simulink model "FullAssemblyMultibody"  (R2025b)
settings: Solver=ode23t  StartTime=0.0  StopTime=16  MaxStep=0.32  RelTol=0.01  AbsTol=1e-3
model workspace: external: MATLAB File E:\Apps\AutodeskInventor\University\MCT333_Design_of_Mechatronics_Systems_1\simscape_multibody_simulation\simulation\FullAssemblyMultibody_DataFile.m (data not in the file)
undefined symbols (not defined in the file or in its folder): smiData, X, Y, Z
libraries: sm_lib x160, Contact_Forces_Lib x46, nesl_utility x5, SignalEditorBlockLib x1
(part 2 of 5)

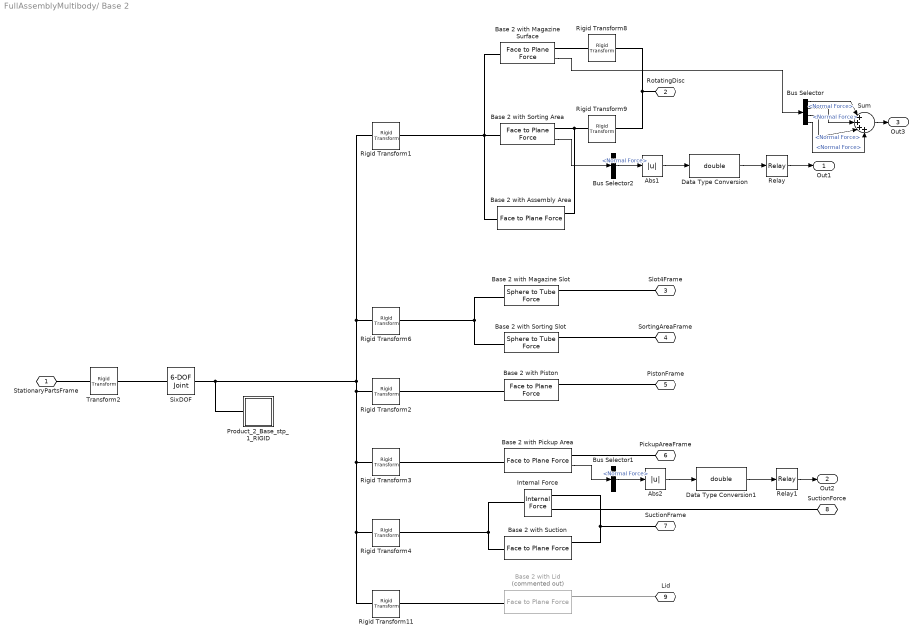
== system FullAssemblyMultibody/ Base 2 ==
  " Base 2 with Piston" : Contact_Forces_Lib/3D/Composite Forces/Face to Plane Force  PlaB_x=0.07  PlaB_y=0.07  PlaB_z=0  FacF_x=0.05  FacF_y=0.05  FacF_z=0.05  FacF_rSph=0.001  force_law_pla2pla=Linear  k_contact_pla2pla=1e4  b_contact_pla2pla=1e4  pen_full_damp_F_pla2pla=1e-4  pen_exponent_pla2pla=1  friction_law_pla2pla=Stick-Slip Continuous  mu_kinetic_pla2pla=0.1  mu_static_pla2pla=0.11  v_thr_pla2pla=0.01  vis_on_pla2pla=off  vis_opc_en_box2box=0  vis_len_plaLz=0.005  vis_clr=[0.9 0.2 0.2]  vis_opc=0.7
      settings: SourceProductName=Simscape Multibody Contact Forces Library
  Abs1 : Abs  SaturateOnIntegerOverflow=off
  Abs2 : Abs  SaturateOnIntegerOverflow=off
  Base 2 with Assembly Area : Contact_Forces_Lib/3D/Composite Forces/Face to Plane Force  PlaB_x=0.1  PlaB_y=0.1  PlaB_z=0  FacF_x=0.05  FacF_y=0.05  FacF_z=0.05  FacF_rSph=0.001  force_law_pla2pla=Linear  k_contact_pla2pla=1e4  b_contact_pla2pla=1e4  pen_full_damp_F_pla2pla=1e-4  pen_exponent_pla2pla=1  friction_law_pla2pla=Stick-Slip Continuous  mu_kinetic_pla2pla=0.1  mu_static_pla2pla=0.11  v_thr_pla2pla=0.01  vis_on_pla2pla=off  vis_opc_en_box2box=0  vis_len_plaLz=0.005  vis_clr=[0.9 0.2 0.2]  vis_opc=0.7
      settings: SourceProductName=Simscape Multibody Contact Forces Library
  Base 2 with Lid : Contact_Forces_Lib/3D/Composite Forces/Face to Plane Force  Commented=on  PlaB_x=0.1  PlaB_y=0.1  PlaB_z=0  FacF_x=0.05  FacF_y=0.05  FacF_z=0.05  FacF_rSph=0.001  force_law_pla2pla=Linear  k_contact_pla2pla=1e4  b_contact_pla2pla=1e4  pen_full_damp_F_pla2pla=1e-4  pen_exponent_pla2pla=1  friction_law_pla2pla=Stick-Slip Continuous  mu_kinetic_pla2pla=0.1  mu_static_pla2pla=0.11  v_thr_pla2pla=0.01  vis_on_pla2pla=off  vis_opc_en_box2box=0  vis_len_plaLz=0.005  vis_clr=[0.9 0.2 0.2]  vis_opc=0.7
      settings: SourceProductName=Simscape Multibody Contact Forces Library
  Base 2 with Magazine Slot : Contact_Forces_Lib/3D/Sphere to Tube Force  radius_sphere=0.05/2  radius_tube=0.070/2  d_tube=0.005  l_tube=.04  active_angle=[-180 180]  force_law=Linear  k_contact=100  b_contact=100  pen_full_damp_F=1e-4  pen_exponent=1  custom_param_1=1  custom_param_2=1  friction_law=Stick-Slip Continuous  mu_kinetic=0.1  mu_static=0.11  v_thr=0.001  vis_on=off  vis_opc_en=0  vis_len_tubBx=0.225*0.02  vis_clr=[0.9 0.2 0.2]  vis_opc=0.7
      settings: SourceProductName=Simscape Multibody Contact Forces Library
  Base 2 with Magazine Surface : Contact_Forces_Lib/3D/Composite Forces/Face to Plane Force  PlaB_x=0.4  PlaB_y=0.4  PlaB_z=0  FacF_x=0.04  FacF_y=0.04  FacF_z=0.05  FacF_rSph=0.001  force_law_pla2pla=Linear  k_contact_pla2pla=1e4  b_contact_pla2pla=1e4  pen_full_damp_F_pla2pla=1e-4  pen_exponent_pla2pla=1  friction_law_pla2pla=Stick-Slip Continuous  mu_kinetic_pla2pla=0.1  mu_static_pla2pla=0.11  v_thr_pla2pla=0.01  vis_on_pla2pla=on  vis_opc_en_box2box=0  vis_len_plaLz=0.005  vis_clr=[0.9 0.2 0.2]  vis_opc=0.7
      settings: SourceProductName=Simscape Multibody Contact Forces Library
  Base 2 with Pickup Area : Contact_Forces_Lib/3D/Composite Forces/Face to Plane Force  PlaB_x=0.1  PlaB_y=0.1  PlaB_z=0  FacF_x=0.05  FacF_y=0.05  FacF_z=0.05  FacF_rSph=0.001  force_law_pla2pla=Linear  k_contact_pla2pla=1e4  b_contact_pla2pla=1e4  pen_full_damp_F_pla2pla=1e-4  pen_exponent_pla2pla=1  friction_law_pla2pla=Stick-Slip Continuous  mu_kinetic_pla2pla=0.1  mu_static_pla2pla=0.11  v_thr_pla2pla=0.01  vis_on_pla2pla=off  vis_opc_en_box2box=0  vis_len_plaLz=0.005  vis_clr=[0.9 0.2 0.2]  vis_opc=0.7
      settings: SourceProductName=Simscape Multibody Contact Forces Library
  Base 2 with Sorting Area : Contact_Forces_Lib/3D/Composite Forces/Face to Plane Force  PlaB_x=1  PlaB_y=1  PlaB_z=0  FacF_x=0.04  FacF_y=0.04  FacF_z=0.05  FacF_rSph=0.001  force_law_pla2pla=Linear  k_contact_pla2pla=1e4  b_contact_pla2pla=1e4  pen_full_damp_F_pla2pla=1e-4  pen_exponent_pla2pla=1  friction_law_pla2pla=Stick-Slip Continuous  mu_kinetic_pla2pla=0.1  mu_static_pla2pla=0.11  v_thr_pla2pla=0.01  vis_on_pla2pla=off  vis_opc_en_box2box=0  vis_len_plaLz=0.005  vis_clr=[0.9 0.2 0.2]  vis_opc=0.7
      settings: SourceProductName=Simscape Multibody Contact Forces Library
  Base 2 with Sorting Slot : Contact_Forces_Lib/3D/Sphere to Tube Force  radius_sphere=0.05/2  radius_tube=0.070/2  d_tube=0.005  l_tube=.1  active_angle=[-180 180]  force_law=Linear  k_contact=100  b_contact=100  pen_full_damp_F=1e-4  pen_exponent=1  custom_param_1=1  custom_param_2=1  friction_law=Stick-Slip Continuous  mu_kinetic=0.1  mu_static=0.11  v_thr=0.001  vis_on=off  vis_opc_en=0  vis_len_tubBx=0.225*0.02  vis_clr=[0.9 0.2 0.2]  vis_opc=0.7
      settings: SourceProductName=Simscape Multibody Contact Forces Library
  Base 2 with Suction : Contact_Forces_Lib/3D/Composite Forces/Face to Plane Force  PlaB_x=0.05  PlaB_y=0.05  PlaB_z=0  FacF_x=0.04  FacF_y=0.04  FacF_z=0.05  FacF_rSph=0.001  force_law_pla2pla=Linear  k_contact_pla2pla=1e4  b_contact_pla2pla=1e4  pen_full_damp_F_pla2pla=1e-4  pen_exponent_pla2pla=1  friction_law_pla2pla=Stick-Slip Continuous  mu_kinetic_pla2pla=0.1  mu_static_pla2pla=0.11  v_thr_pla2pla=0.01  vis_on_pla2pla=off  vis_opc_en_box2box=0  vis_len_plaLz=0.005  vis_clr=[0.9 0.2 0.2]  vis_opc=0.7
      settings: SourceProductName=Simscape Multibody Contact Forces Library
  Bus Selector : BusSelector  OutputSignals=fz1.Normal Force,fz2.Normal Force,fz3.Normal Force,fz4.Normal Force
  Bus Selector1 : BusSelector  OutputSignals=fz1.Normal Force
  Bus Selector2 : BusSelector  OutputSignals=fz1.Normal Force
  Data Type Conversion : DataTypeConversion  OutDataTypeStr=double  SaturateOnIntegerOverflow=off  RndMeth=Floor
  Data Type Conversion1 : DataTypeConversion  OutDataTypeStr=double  SaturateOnIntegerOverflow=off  RndMeth=Floor
  Internal Force : sm_lib/Forces and Torques/Internal Force
  Product_2_Base_stp_1_RIGID : Subsystem
  Relay : Relay  OnSwitchValue=0.5  OffSwitchValue=0.005
  Relay1 : Relay  OnSwitchValue=0.5  OffSwitchValue=0.005
  Rigid Transform1 : sm_lib/Frames and Transforms/Rigid Transform  RotationMethod=StandardAxis  FollAlignAxisA=+X  BaseAlignAxisA=+Y  FollAlignAxisB=+Y  BaseAlignAxisB=+Z  RotationStandardAxis=+X  RotationAngle=90  RotationAngleUnits=deg  RotationArbitraryAxis=[0 0 1]  RotationSequenceAxes=FollowerAxes  RotationSequence=XYX  RotationSequenceAngles=[0 0 0]  RotationSequenceAnglesUnits=deg  RotationMatrix=[1 0 0;0 1 0;0 0 1]  Quaternion=[1 0 0 0]  TranslationMethod=StandardAxis  TranslationCartesianOffset=[0 0 0]  TranslationCartesianOffsetUnits=m  TranslationStandardAxis=-Y  TranslationStandardOffset=40  TranslationStandardOffsetUnits=mm  TranslationROffset=0  TranslationROffsetUnits=m  TranslationThetaOffset=0  TranslationThetaOffsetUnits=deg  TranslationZOffset=0  TranslationZOffsetUnits=m
  Rigid Transform11 : sm_lib/Frames and Transforms/Rigid Transform  RotationMethod=StandardAxis  FollAlignAxisA=+X  BaseAlignAxisA=+Y  FollAlignAxisB=+Y  BaseAlignAxisB=+Z  RotationStandardAxis=+X  RotationAngle=90  RotationAngleUnits=deg  RotationArbitraryAxis=[0 0 1]  RotationSequenceAxes=FollowerAxes  RotationSequence=XYX  RotationSequenceAngles=[0 0 0]  RotationSequenceAnglesUnits=deg  RotationMatrix=[1 0 0;0 1 0;0 0 1]  Quaternion=[1 0 0 0]  TranslationMethod=StandardAxis  TranslationCartesianOffset=[0 20 50]  TranslationCartesianOffsetUnits=mm  TranslationStandardAxis=-Y  TranslationStandardOffset=20  TranslationStandardOffsetUnits=mm  TranslationROffset=0  TranslationROffsetUnits=m  TranslationThetaOffset=0  TranslationThetaOffsetUnits=deg  TranslationZOffset=0  TranslationZOffsetUnits=m
  Rigid Transform2 : sm_lib/Frames and Transforms/Rigid Transform  RotationMethod=None  FollAlignAxisA=+X  BaseAlignAxisA=+Y  FollAlignAxisB=+Y  BaseAlignAxisB=+Z  RotationStandardAxis=+Z  RotationAngle=0  RotationAngleUnits=deg  RotationArbitraryAxis=[0 0 1]  RotationSequenceAxes=FollowerAxes  RotationSequence=XYX  RotationSequenceAngles=[0 0 0]  RotationSequenceAnglesUnits=deg  RotationMatrix=[1 0 0;0 1 0;0 0 1]  Quaternion=[1 0 0 0]  TranslationMethod=Cartesian  TranslationCartesianOffset=[0 20 50]  TranslationCartesianOffsetUnits=mm  TranslationStandardAxis=+Y  TranslationStandardOffset=50  TranslationStandardOffsetUnits=mm  TranslationROffset=0  TranslationROffsetUnits=m  TranslationThetaOffset=0  TranslationThetaOffsetUnits=deg  TranslationZOffset=0  TranslationZOffsetUnits=m
  Rigid Transform3 : sm_lib/Frames and Transforms/Rigid Transform  RotationMethod=None  FollAlignAxisA=+X  BaseAlignAxisA=+Y  FollAlignAxisB=+Y  BaseAlignAxisB=+Z  RotationStandardAxis=+X  RotationAngle=90  RotationAngleUnits=deg  RotationArbitraryAxis=[0 0 1]  RotationSequenceAxes=FollowerAxes  RotationSequence=XYX  RotationSequenceAngles=[0 0 0]  RotationSequenceAnglesUnits=deg  RotationMatrix=[1 0 0;0 1 0;0 0 1]  Quaternion=[1 0 0 0]  TranslationMethod=Cartesian  TranslationCartesianOffset=[0 20 50]  TranslationCartesianOffsetUnits=mm  TranslationStandardAxis=+Y  TranslationStandardOffset=50  TranslationStandardOffsetUnits=mm  TranslationROffset=0  TranslationROffsetUnits=m  TranslationThetaOffset=0  TranslationThetaOffsetUnits=deg  TranslationZOffset=0  TranslationZOffsetUnits=m
  Rigid Transform4 : sm_lib/Frames and Transforms/Rigid Transform  RotationMethod=StandardAxis  FollAlignAxisA=+X  BaseAlignAxisA=+Y  FollAlignAxisB=+Y  BaseAlignAxisB=+Z  RotationStandardAxis=+X  RotationAngle=90  RotationAngleUnits=deg  RotationArbitraryAxis=[0 0 1]  RotationSequenceAxes=FollowerAxes  RotationSequence=XYX  RotationSequenceAngles=[0 0 0]  RotationSequenceAnglesUnits=deg  RotationMatrix=[1 0 0;0 1 0;0 0 1]  Quaternion=[1 0 0 0]  TranslationMethod=StandardAxis  TranslationCartesianOffset=[0 20 50]  TranslationCartesianOffsetUnits=mm  TranslationStandardAxis=-Y  TranslationStandardOffset=10  TranslationStandardOffsetUnits=mm  TranslationROffset=0  TranslationROffsetUnits=m  TranslationThetaOffset=0  TranslationThetaOffsetUnits=deg  TranslationZOffset=0  TranslationZOffsetUnits=m
  Rigid Transform6 : sm_lib/Frames and Transforms/Rigid Transform  RotationMethod=None  FollAlignAxisA=+X  BaseAlignAxisA=+Y  FollAlignAxisB=+Y  BaseAlignAxisB=+Z  RotationStandardAxis=+Z  RotationAngle=0  RotationAngleUnits=deg  RotationArbitraryAxis=[0 0 1]  RotationSequenceAxes=FollowerAxes  RotationSequence=XYX  RotationSequenceAngles=[0 0 0]  RotationSequenceAnglesUnits=deg  RotationMatrix=[1 0 0;0 1 0;0 0 1]  Quaternion=[1 0 0 0]  TranslationMethod=StandardAxis  TranslationCartesianOffset=[0 0 0]  TranslationCartesianOffsetUnits=m  TranslationStandardAxis=+Y  TranslationStandardOffset=15  TranslationStandardOffsetUnits=mm  TranslationROffset=0  TranslationROffsetUnits=m  TranslationThetaOffset=0  TranslationThetaOffsetUnits=deg  TranslationZOffset=0  TranslationZOffsetUnits=m
  Rigid Transform8 : sm_lib/Frames and Transforms/Rigid Transform  RotationMethod=None  FollAlignAxisA=+X  BaseAlignAxisA=+Y  FollAlignAxisB=+Y  BaseAlignAxisB=+Z  RotationStandardAxis=+Z  RotationAngle=0  RotationAngleUnits=deg  RotationArbitraryAxis=[0 0 1]  RotationSequenceAxes=FollowerAxes  RotationSequence=XYX  RotationSequenceAngles=[0 0 0]  RotationSequenceAnglesUnits=deg  RotationMatrix=[1 0 0;0 1 0;0 0 1]  Quaternion=[1 0 0 0]  TranslationMethod=StandardAxis  TranslationCartesianOffset=[0 0 0]  TranslationCartesianOffsetUnits=m  TranslationStandardAxis=-X  TranslationStandardOffset=225  TranslationStandardOffsetUnits=mm  TranslationROffset=0  TranslationROffsetUnits=m  TranslationThetaOffset=0  TranslationThetaOffsetUnits=deg  TranslationZOffset=0  TranslationZOffsetUnits=m
  Rigid Transform9 : sm_lib/Frames and Transforms/Rigid Transform  RotationMethod=None  FollAlignAxisA=+X  BaseAlignAxisA=+Y  FollAlignAxisB=+Y  BaseAlignAxisB=+Z  RotationStandardAxis=+Z  RotationAngle=0  RotationAngleUnits=deg  RotationArbitraryAxis=[0 0 1]  RotationSequenceAxes=FollowerAxes  RotationSequence=XYX  RotationSequenceAngles=[0 0 0]  RotationSequenceAnglesUnits=deg  RotationMatrix=[1 0 0;0 1 0;0 0 1]  Quaternion=[1 0 0 0]  TranslationMethod=StandardAxis  TranslationCartesianOffset=[0 0 0]  TranslationCartesianOffsetUnits=m  TranslationStandardAxis=+Z  TranslationStandardOffset=120  TranslationStandardOffsetUnits=mm  TranslationROffset=0  TranslationROffsetUnits=m  TranslationThetaOffset=0  TranslationThetaOffsetUnits=deg  TranslationZOffset=0  TranslationZOffsetUnits=m
  SixDOF : sm_lib/Joints/6-DOF Joint  JointMode=Normal  CompositeWrenchDir=FollowerOnBase  CompositeWrenchFrame=BaseFrame  SenseConstraintForce=off  SenseConstraintTorque=off  SenseTotalForce=off  SenseTotalTorque=off  PxPositionTargetSpecify=off  PxPositionTargetPriority=High  PxPositionTargetValue=0  PxPositionTargetValueUnits=m  PxVelocityTargetSpecify=off  PxVelocityTargetPriority=High  PxVelocityTargetValue=0  PxVelocityTargetValueUnits=m/s  PxEquilibriumPosition=0  PxEquilibriumPositionUnits=m  PxSpringStiffness=0  PxSpringStiffnessUnits=N/m  PxDampingCoefficient=0  PxDampingCoefficientUnits=N/(m/s)  PxLowerLimitSpecify=off  PxLowerLimitBound=-1  PxLowerLimitBoundUnits=m  PxLowerLimitStiffness=1e6  PxLowerLimitStiffnessUnits=N/m  PxLowerLimitDamping=1e3  PxLowerLimitDampingUnits=N/(m/s)  PxLowerLimitTransitionRegionWidth=1e-4  PxLowerLimitTransitionRegionWidthUnits=m  PxUpperLimitSpecify=off  PxUpperLimitBound=1  PxUpperLimitBoundUnits=m  PxUpperLimitStiffness=1e6  PxUpperLimitStiffnessUnits=N/m  PxUpperLimitDamping=1e3  PxUpperLimitDampingUnits=N/(m/s)  PxUpperLimitTransitionRegionWidth=1e-4  PxUpperLimitTransitionRegionWidthUnits=m  PxTorqueActuationMode=NoTorque  PxMotionActuationMode=ComputedMotion  PxSensePosition=off  PxSenseVelocity=off  PxSenseAcceleration=off  PxSenseTorqueForce=off  PxSenseLowerLimitTorqueForce=off  PxSenseUpperLimitTorqueForce=off  PyPositionTargetSpecify=on  PyPositionTargetPriority=High  PyPositionTargetValue=30  PyPositionTargetValueUnits=mm  PyVelocityTargetSpecify=off  PyVelocityTargetPriority=High  PyVelocityTargetValue=0  PyVelocityTargetValueUnits=m/s  PyEquilibriumPosition=0  PyEquilibriumPositionUnits=m  PySpringStiffness=0  PySpringStiffnessUnits=N/m  PyDampingCoefficient=0  PyDampingCoefficientUnits=N/(m/s)  PyLowerLimitSpecify=off  PyLowerLimitBound=-1  PyLowerLimitBoundUnits=m  PyLowerLimitStiffness=1e6  PyLowerLimitStiffnessUnits=N/m  PyLowerLimitDamping=1e3  PyLowerLimitDampingUnits=N/(m/s)  PyLowerLimitTransitionRegionWidth=1e-4  PyLowerLimitTransitionRegionWidthUnits=m  PyUpperLimitSpecify=off  PyUpperLimitBound=1  PyUpperLimitBoundUnits=m  PyUpperLimitStiffness=1e6  PyUpperLimitStiffnessUnits=N/m  PyUpperLimitDamping=1e3  PyUpperLimitDampingUnits=N/(m/s)  PyUpperLimitTransitionRegionWidth=1e-4  PyUpperLimitTransitionRegionWidthUnits=m  PyTorqueActuationMode=NoTorque  PyMotionActuationMode=ComputedMotion  PySensePosition=off  PySenseVelocity=off  PySenseAcceleration=off  PySenseTorqueForce=off  PySenseLowerLimitTorqueForce=off  PySenseUpperLimitTorqueForce=off  PzPositionTargetSpecify=off  PzPositionTargetPriority=High  PzPositionTargetValue=0  PzPositionTargetValueUnits=m  PzVelocityTargetSpecify=off  PzVelocityTargetPriority=High  PzVelocityTargetValue=0  PzVelocityTargetValueUnits=m/s  PzEquilibriumPosition=0  PzEquilibriumPositionUnits=m  PzSpringStiffness=0  PzSpringStiffnessUnits=N/m  PzDampingCoefficient=0  PzDampingCoefficientUnits=N/(m/s)  PzLowerLimitSpecify=off  PzLowerLimitBound=-1  PzLowerLimitBoundUnits=m  PzLowerLimitStiffness=1e6  PzLowerLimitStiffnessUnits=N/m  PzLowerLimitDamping=1e3  PzLowerLimitDampingUnits=N/(m/s)  PzLowerLimitTransitionRegionWidth=1e-4  PzLowerLimitTransitionRegionWidthUnits=m  PzUpperLimitSpecify=off  PzUpperLimitBound=1  PzUpperLimitBoundUnits=m  PzUpperLimitStiffness=1e6  PzUpperLimitStiffnessUnits=N/m  PzUpperLimitDamping=1e3  PzUpperLimitDampingUnits=N/(m/s)  PzUpperLimitTransitionRegionWidth=1e-4  PzUpperLimitTransitionRegionWidthUnits=m  PzTorqueActuationMode=NoTorque  PzMotionActuationMode=ComputedMotion  PzSensePosition=off  PzSenseVelocity=off  PzSenseAcceleration=off  PzSenseTorqueForce=off  PzSenseLowerLimitTorqueForce=off  PzSenseUpperLimitTorqueForce=off  SphPositionTargetSpecify=off  SphPositionTargetPriority=High  SphPositionTargetRotationMethod=None  SphPositionTargetFollAlignAxisA=+X  SphPositionTargetBaseAlignAxisA=+Y  SphPositionTargetFollAlignAxisB=+Y  SphPositionTargetBaseAlignAxisB=+Z  SphPositionTargetRotationStandardAxis=+Z  SphPositionTargetRotationAngle=0  SphPositionTargetRotationAngleUnits=deg  SphPositionTargetRotationArbitraryAxis=[0 0 1]  SphPositionTargetRotationSequenceAxes=FollowerAxes  SphPositionTargetRotationSequence=XYX  SphPositionTargetRotationSequenceAngles=[0 0 0]  SphPositionTargetRotationSequenceAnglesUnits=deg  SphPositionTargetRotationMatrix=[1 0 0;0 1 0;0 0 1]  SphPositionTargetQuaternion=[1 0 0 0]  SphVelocityTargetSpecify=off  SphVelocityTargetPriority=High  SphVelocityTargetValue=[0 0 0]  SphVelocityTargetValueUnits=deg/s  SphVelocityTargetInFollowerFrame=on  SphEqPosRotationMethod=None  SphEqPosFollAlignAxisA=+X  SphEqPosBaseAlignAxisA=+Y  SphEqPosFollAlignAxisB=+Y  SphEqPosBaseAlignAxisB=+Z  SphEqPosRotationStandardAxis=+Z  SphEqPosRotationAngle=0  SphEqPosRotationAngleUnits=deg  SphEqPosRotationArbitraryAxis=[0 0 1]  SphEqPosRotationSequenceAxes=FollowerAxes  SphEqPosRotationSequence=XYX  SphEqPosRotationSequenceAngles=[0 0 0]  SphEqPosRotationSequenceAnglesUnits=deg  SphEqPosRotationMatrix=[1 0 0;0 1 0;0 0 1]  SphEqPosQuaternion=[1 0 0 0]  SphSpringStiffness=0  SphSpringStiffnessUnits=N*m/deg  SphDampingCoefficient=0  SphDampingCoefficientUnits=N*m/(deg/s)  SphLowerLimitSpecify=off  SphLowerLimitBound=15  SphLowerLimitBoundUnits=deg  SphLowerLimitStiffness=1e4  SphLowerLimitStiffnessUnits=N*m/deg  SphLowerLimitDamping=10  SphLowerLimitDampingUnits=N*m/(deg/s)  SphLowerLimitTransitionRegionWidth=0.1  SphLowerLimitTransitionRegionWidthUnits=deg  SphUpperLimitSpecify=off  SphUpperLimitBound=45  SphUpperLimitBoundUnits=deg  SphUpperLimitStiffness=1e4  SphUpperLimitStiffnessUnits=N*m/deg  SphUpperLimitDamping=10  SphUpperLimitDampingUnits=N*m/(deg/s)  SphUpperLimitTransitionRegionWidth=0.1  SphUpperLimitTransitionRegionWidthUnits=deg  SphTorqueActuationMode=NoTorque  SphActuateTorqueX=off  SphActuateTorqueY=off  SphActuateTorqueZ=off  SphActuateTorque=off  SphActuationFrame=BaseFrame  SphSensePosition=off  SphSenseVelocityX=off  SphSenseVelocityY=off  SphSenseVelocityZ=off  SphSenseVelocity=off  SphSenseAccelerationX=off  SphSenseAccelerationY=off  SphSenseAccelerationZ=off  SphSenseAcceleration=off  SphSenseLowerLimitTorqueMag=off  SphSenseUpperLimitTorqueMag=off  SphSensingFrame=FollowerFrame
  Sum : Sum  Inputs=|++++
  Transform2 : sm_lib/Frames and Transforms/Rigid Transform  RotationMethod=ArbitraryAxis  FollAlignAxisA=+X  BaseAlignAxisA=+Y  FollAlignAxisB=+Y  BaseAlignAxisB=+Z  RotationStandardAxis=+Z  RotationAngle=smiData.RigidTransform(31).angle  RotationAngleUnits=rad  RotationArbitraryAxis=smiData.RigidTransform(31).axis  RotationSequenceAxes=FollowerAxes  RotationSequence=XYX  RotationSequenceAngles=[0 0 0]  RotationSequenceAnglesUnits=deg  RotationMatrix=[1 0 0;0 1 0;0 0 1]  Quaternion=[1 0 0 0]  TranslationMethod=Cartesian  TranslationCartesianOffset=smiData.RigidTransform(31).translation  TranslationCartesianOffsetUnits=mm  TranslationStandardAxis=+Z  TranslationStandardOffset=0  TranslationStandardOffsetUnits=m  TranslationROffset=0  TranslationROffsetUnits=m  TranslationThetaOffset=0  TranslationThetaOffsetUnits=deg  TranslationZOffset=0  TranslationZOffsetUnits=m
  StationaryPartsFrame : PMIOPort  Side=Left
  RotatingDisc : PMIOPort  Port=2  Side=Left
  Slot4Frame : PMIOPort  Port=3  Side=Left
  SortingAreaFrame : PMIOPort  Port=4  Side=Left
  PistonFrame : PMIOPort  Port=5  Side=Left
  PickupAreaFrame : PMIOPort  Port=6  Side=Left
  SuctionFrame : PMIOPort  Port=7  Side=Left
  " SuctionForce" : PMIOPort  Port=8  Side=Left
  Lid : PMIOPort  Port=9  Side=Left
  Out1 : Outport
  Out2 : Outport  Port=2
  Out3 : Outport  Port=3
  wires:
  Base 2 with Pickup Area/1 -> Bus Selector1/1
  Base 2 with Sorting Area/1 -> Bus Selector2/1
  Bus Selector2/1 -> Abs1/1  "<Normal Force>"
  Abs1/1 -> Data Type Conversion/1
  Relay/1 -> Out1/1
  Data Type Conversion/1 -> Relay/1
  Bus Selector1/1 -> Abs2/1  "<Normal Force>"
  Abs2/1 -> Data Type Conversion1/1
  Data Type Conversion1/1 -> Relay1/1
  Relay1/1 -> Out2/1
  Base 2 with Magazine Surface/1 -> Bus Selector/1
  Sum/1 -> Out3/1
  Bus Selector/2 -> Sum/2  "<Normal Force>"
  Bus Selector/4 -> Sum/4  "<Normal Force>"
  Bus Selector/1 -> Sum/1  "<Normal Force>"
  Bus Selector/3 -> Sum/3  "<Normal Force>"
  connections:
  Base 2 with Sorting Slot/RConn1 -- SortingAreaFrame/RConn1
  Transform2/LConn1 -- StationaryPartsFrame/RConn1
  Slot4Frame/RConn1 -- Base 2 with Magazine Slot/RConn1
  Rigid Transform8/LConn1 -- RotatingDisc/RConn1 -- Rigid Transform9/LConn1
  Base 2 with Sorting Area/RConn1 -- Rigid Transform9/RConn1 -- Base 2 with Assembly Area/RConn1
  Base 2 with Magazine Slot/LConn1 -- Rigid Transform6/RConn1 -- Base 2 with Sorting Slot/LConn1
  Base 2 with Magazine Surface/RConn1 -- Rigid Transform8/RConn1
  Rigid Transform11/LConn1 -- Rigid Transform4/LConn1 -- Rigid Transform3/LConn1 -- Rigid Transform2/LConn1 -- Rigid Transform6/LConn1 -- Rigid Transform1/LConn1 -- Product_2_Base_stp_1_RIGID/LConn1 -- SixDOF/RConn1
  Transform2/RConn1 -- SixDOF/LConn1
  " Base 2 with Piston"/RConn1 -- PistonFrame/RConn1
  Rigid Transform3/RConn1 -- Base 2 with Pickup Area/LConn1
  PickupAreaFrame/RConn1 -- Base 2 with Pickup Area/RConn1
  Rigid Transform2/RConn1 -- " Base 2 with Piston"/LConn1
  Rigid Transform4/RConn1 -- Base 2 with Suction/LConn1 -- Internal Force/RConn1
  Base 2 with Suction/RConn1 -- SuctionFrame/RConn1 -- Internal Force/LConn1
  Rigid Transform11/RConn1 -- Base 2 with Lid/LConn1
  Base 2 with Lid/RConn1 -- Lid/RConn1
  " SuctionForce"/RConn1 -- Internal Force/LConn2
  Base 2 with Magazine Surface/LConn1 -- Rigid Transform1/RConn1 -- Base 2 with Sorting Area/LConn1 -- Base 2 with Assembly Area/LConn1

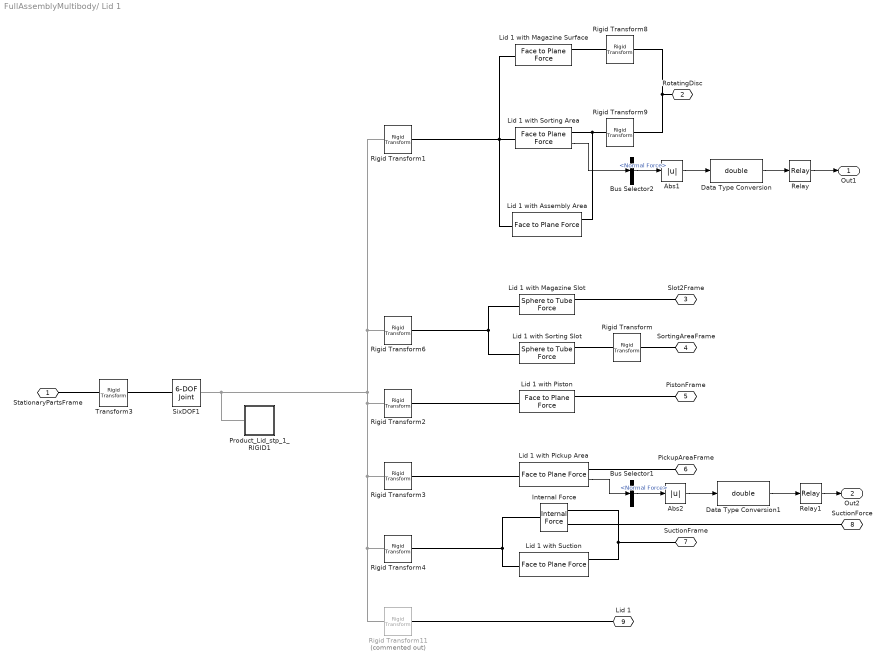
== system FullAssemblyMultibody/ Lid 1 ==
  " Lid 1 with Piston" : Contact_Forces_Lib/3D/Composite Forces/Face to Plane Force  PlaB_x=0.07  PlaB_y=0.07  PlaB_z=0  FacF_x=0.05  FacF_y=0.05  FacF_z=0.05  FacF_rSph=0.001  force_law_pla2pla=Linear  k_contact_pla2pla=1e4  b_contact_pla2pla=1e4  pen_full_damp_F_pla2pla=1e-4  pen_exponent_pla2pla=1  friction_law_pla2pla=Stick-Slip Continuous  mu_kinetic_pla2pla=0.1  mu_static_pla2pla=0.11  v_thr_pla2pla=0.01  vis_on_pla2pla=off  vis_opc_en_box2box=0  vis_len_plaLz=0.005  vis_clr=[0.9 0.2 0.2]  vis_opc=0.7
      settings: SourceProductName=Simscape Multibody Contact Forces Library
  Abs1 : Abs  SaturateOnIntegerOverflow=off
  Abs2 : Abs  SaturateOnIntegerOverflow=off
  Bus Selector1 : BusSelector  OutputSignals=fz1.Normal Force
  Bus Selector2 : BusSelector  OutputSignals=fz1.Normal Force
  Data Type Conversion : DataTypeConversion  OutDataTypeStr=double  SaturateOnIntegerOverflow=off  RndMeth=Floor
  Data Type Conversion1 : DataTypeConversion  OutDataTypeStr=double  SaturateOnIntegerOverflow=off  RndMeth=Floor
  Internal Force : sm_lib/Forces and Torques/Internal Force
  Lid 1 with Assembly Area : Contact_Forces_Lib/3D/Composite Forces/Face to Plane Force  PlaB_x=0.1  PlaB_y=0.1  PlaB_z=0  FacF_x=0.05  FacF_y=0.05  FacF_z=0.05  FacF_rSph=0.001  force_law_pla2pla=Linear  k_contact_pla2pla=1e4  b_contact_pla2pla=1e4  pen_full_damp_F_pla2pla=1e-4  pen_exponent_pla2pla=1  friction_law_pla2pla=Stick-Slip Continuous  mu_kinetic_pla2pla=0.1  mu_static_pla2pla=0.11  v_thr_pla2pla=0.01  vis_on_pla2pla=off  vis_opc_en_box2box=0  vis_len_plaLz=0.005  vis_clr=[0.9 0.2 0.2]  vis_opc=0.7
      settings: SourceProductName=Simscape Multibody Contact Forces Library
  Lid 1 with Magazine Slot : Contact_Forces_Lib/3D/Sphere to Tube Force  radius_sphere=0.05/2  radius_tube=0.070/2  d_tube=0.005  l_tube=.04  active_angle=[-180 180]  force_law=Linear  k_contact=100  b_contact=100  pen_full_damp_F=1e-4  pen_exponent=1  custom_param_1=1  custom_param_2=1  friction_law=Stick-Slip Continuous  mu_kinetic=0.1  mu_static=0.11  v_thr=0.001  vis_on=off  vis_opc_en=0  vis_len_tubBx=0.225*0.02  vis_clr=[0.9 0.2 0.2]  vis_opc=0.7
      settings: SourceProductName=Simscape Multibody Contact Forces Library
  Lid 1 with Magazine Surface : Contact_Forces_Lib/3D/Composite Forces/Face to Plane Force  PlaB_x=0.4  PlaB_y=0.4  PlaB_z=0  FacF_x=0.04  FacF_y=0.04  FacF_z=0.05  FacF_rSph=0.001  force_law_pla2pla=Linear  k_contact_pla2pla=1e4  b_contact_pla2pla=1e4  pen_full_damp_F_pla2pla=1e-4  pen_exponent_pla2pla=1  friction_law_pla2pla=Stick-Slip Continuous  mu_kinetic_pla2pla=0.1  mu_static_pla2pla=0.11  v_thr_pla2pla=0.01  vis_on_pla2pla=off  vis_opc_en_box2box=0  vis_len_plaLz=0.005  vis_clr=[0.9 0.2 0.2]  vis_opc=0.7
      settings: SourceProductName=Simscape Multibody Contact Forces Library
  Lid 1 with Pickup Area : Contact_Forces_Lib/3D/Composite Forces/Face to Plane Force  PlaB_x=0.1  PlaB_y=0.1  PlaB_z=0  FacF_x=0.05  FacF_y=0.05  FacF_z=0.05  FacF_rSph=0.001  force_law_pla2pla=Linear  k_contact_pla2pla=1e4  b_contact_pla2pla=1e4  pen_full_damp_F_pla2pla=1e-4  pen_exponent_pla2pla=1  friction_law_pla2pla=Stick-Slip Continuous  mu_kinetic_pla2pla=0.1  mu_static_pla2pla=0.11  v_thr_pla2pla=0.01  vis_on_pla2pla=off  vis_opc_en_box2box=0  vis_len_plaLz=0.005  vis_clr=[0.9 0.2 0.2]  vis_opc=0.7
      settings: SourceProductName=Simscape Multibody Contact Forces Library
  Lid 1 with Sorting Area : Contact_Forces_Lib/3D/Composite Forces/Face to Plane Force  PlaB_x=1  PlaB_y=1  PlaB_z=0  FacF_x=0.04  FacF_y=0.04  FacF_z=0.05  FacF_rSph=0.001  force_law_pla2pla=Linear  k_contact_pla2pla=1e4  b_contact_pla2pla=1e4  pen_full_damp_F_pla2pla=1e-4  pen_exponent_pla2pla=1  friction_law_pla2pla=Stick-Slip Continuous  mu_kinetic_pla2pla=0.1  mu_static_pla2pla=0.11  v_thr_pla2pla=0.01  vis_on_pla2pla=off  vis_opc_en_box2box=0  vis_len_plaLz=0.005  vis_clr=[0.9 0.2 0.2]  vis_opc=0.7
      settings: SourceProductName=Simscape Multibody Contact Forces Library
  Lid 1 with Sorting Slot : Contact_Forces_Lib/3D/Sphere to Tube Force  radius_sphere=0.05/2  radius_tube=0.055/2  d_tube=0.005  l_tube=.11  active_angle=[-180 180]  force_law=Linear  k_contact=100  b_contact=100  pen_full_damp_F=1e-4  pen_exponent=1  custom_param_1=1  custom_param_2=1  friction_law=Stick-Slip Continuous  mu_kinetic=0.1  mu_static=0.11  v_thr=0.001  vis_on=off  vis_opc_en=0  vis_len_tubBx=0.225*0.02  vis_clr=[0.9 0.2 0.2]  vis_opc=0.7
      settings: SourceProductName=Simscape Multibody Contact Forces Library
  Lid 1 with Suction : Contact_Forces_Lib/3D/Composite Forces/Face to Plane Force  PlaB_x=0.05  PlaB_y=0.05  PlaB_z=0  FacF_x=0.04  FacF_y=0.04  FacF_z=0.05  FacF_rSph=0.001  force_law_pla2pla=Linear  k_contact_pla2pla=1e4  b_contact_pla2pla=1e4  pen_full_damp_F_pla2pla=1e-4  pen_exponent_pla2pla=1  friction_law_pla2pla=Stick-Slip Continuous  mu_kinetic_pla2pla=0.1  mu_static_pla2pla=0.11  v_thr_pla2pla=0.01  vis_on_pla2pla=off  vis_opc_en_box2box=0  vis_len_plaLz=0.005  vis_clr=[0.9 0.2 0.2]  vis_opc=0.7
      settings: SourceProductName=Simscape Multibody Contact Forces Library
  Product_Lid_stp_1_RIGID1 : Subsystem
  Relay : Relay  OnSwitchValue=0.5  OffSwitchValue=0.005
  Relay1 : Relay  OnSwitchValue=0.5  OffSwitchValue=0.005
  Rigid Transform : sm_lib/Frames and Transforms/Rigid Transform  RotationMethod=None  FollAlignAxisA=+X  BaseAlignAxisA=+Y  FollAlignAxisB=+Y  BaseAlignAxisB=+Z  RotationStandardAxis=+Z  RotationAngle=0  RotationAngleUnits=deg  RotationArbitraryAxis=[0 0 1]  RotationSequenceAxes=FollowerAxes  RotationSequence=XYX  RotationSequenceAngles=[0 0 0]  RotationSequenceAnglesUnits=deg  RotationMatrix=[1 0 0;0 1 0;0 0 1]  Quaternion=[1 0 0 0]  TranslationMethod=StandardAxis  TranslationCartesianOffset=[0 0 0]  TranslationCartesianOffsetUnits=m  TranslationStandardAxis=+Z  TranslationStandardOffset=20  TranslationStandardOffsetUnits=mm  TranslationROffset=0  TranslationROffsetUnits=m  TranslationThetaOffset=0  TranslationThetaOffsetUnits=deg  TranslationZOffset=0  TranslationZOffsetUnits=m
  Rigid Transform1 : sm_lib/Frames and Transforms/Rigid Transform  RotationMethod=StandardAxis  FollAlignAxisA=+X  BaseAlignAxisA=+Y  FollAlignAxisB=+Y  BaseAlignAxisB=+Z  RotationStandardAxis=+X  RotationAngle=90  RotationAngleUnits=deg  RotationArbitraryAxis=[0 0 1]  RotationSequenceAxes=FollowerAxes  RotationSequence=XYX  RotationSequenceAngles=[0 0 0]  RotationSequenceAnglesUnits=deg  RotationMatrix=[1 0 0;0 1 0;0 0 1]  Quaternion=[1 0 0 0]  TranslationMethod=StandardAxis  TranslationCartesianOffset=[0 0 0]  TranslationCartesianOffsetUnits=m  TranslationStandardAxis=-Y  TranslationStandardOffset=40  TranslationStandardOffsetUnits=mm  TranslationROffset=0  TranslationROffsetUnits=m  TranslationThetaOffset=0  TranslationThetaOffsetUnits=deg  TranslationZOffset=0  TranslationZOffsetUnits=m
  Rigid Transform11 : sm_lib/Frames and Transforms/Rigid Transform  Commented=on  RotationMethod=StandardAxis  FollAlignAxisA=+X  BaseAlignAxisA=+Y  FollAlignAxisB=+Y  BaseAlignAxisB=+Z  RotationStandardAxis=+X  RotationAngle=90  RotationAngleUnits=deg  RotationArbitraryAxis=[0 0 1]  RotationSequenceAxes=FollowerAxes  RotationSequence=XYX  RotationSequenceAngles=[0 0 0]  RotationSequenceAnglesUnits=deg  RotationMatrix=[1 0 0;0 1 0;0 0 1]  Quaternion=[1 0 0 0]  TranslationMethod=StandardAxis  TranslationCartesianOffset=[0 20 50]  TranslationCartesianOffsetUnits=mm  TranslationStandardAxis=-Y  TranslationStandardOffset=20  TranslationStandardOffsetUnits=mm  TranslationROffset=0  TranslationROffsetUnits=m  TranslationThetaOffset=0  TranslationThetaOffsetUnits=deg  TranslationZOffset=0  TranslationZOffsetUnits=m
  Rigid Transform2 : sm_lib/Frames and Transforms/Rigid Transform  RotationMethod=StandardAxis  FollAlignAxisA=+X  BaseAlignAxisA=+Y  FollAlignAxisB=+Y  BaseAlignAxisB=+Z  RotationStandardAxis=+Z  RotationAngle=90  RotationAngleUnits=deg  RotationArbitraryAxis=[0 0 1]  RotationSequenceAxes=FollowerAxes  RotationSequence=XYX  RotationSequenceAngles=[0 0 0]  RotationSequenceAnglesUnits=deg  RotationMatrix=[1 0 0;0 1 0;0 0 1]  Quaternion=[1 0 0 0]  TranslationMethod=Cartesian  TranslationCartesianOffset=[0 20 70]  TranslationCartesianOffsetUnits=mm  TranslationStandardAxis=+Y  TranslationStandardOffset=50  TranslationStandardOffsetUnits=mm  TranslationROffset=0  TranslationROffsetUnits=m  TranslationThetaOffset=0  TranslationThetaOffsetUnits=deg  TranslationZOffset=0  TranslationZOffsetUnits=m
  Rigid Transform3 : sm_lib/Frames and Transforms/Rigid Transform  RotationMethod=None  FollAlignAxisA=+X  BaseAlignAxisA=+Y  FollAlignAxisB=+Y  BaseAlignAxisB=+Z  RotationStandardAxis=+X  RotationAngle=90  RotationAngleUnits=deg  RotationArbitraryAxis=[0 0 1]  RotationSequenceAxes=FollowerAxes  RotationSequence=XYX  RotationSequenceAngles=[0 0 0]  RotationSequenceAnglesUnits=deg  RotationMatrix=[1 0 0;0 1 0;0 0 1]  Quaternion=[1 0 0 0]  TranslationMethod=Cartesian  TranslationCartesianOffset=[0 20 50]  TranslationCartesianOffsetUnits=mm  TranslationStandardAxis=+Y  TranslationStandardOffset=50  TranslationStandardOffsetUnits=mm  TranslationROffset=0  TranslationROffsetUnits=m  TranslationThetaOffset=0  TranslationThetaOffsetUnits=deg  TranslationZOffset=0  TranslationZOffsetUnits=m
  Rigid Transform4 : sm_lib/Frames and Transforms/Rigid Transform  RotationMethod=StandardAxis  FollAlignAxisA=+X  BaseAlignAxisA=+Y  FollAlignAxisB=+Y  BaseAlignAxisB=+Z  RotationStandardAxis=+X  RotationAngle=90  RotationAngleUnits=deg  RotationArbitraryAxis=[0 0 1]  RotationSequenceAxes=FollowerAxes  RotationSequence=XYX  RotationSequenceAngles=[0 0 0]  RotationSequenceAnglesUnits=deg  RotationMatrix=[1 0 0;0 1 0;0 0 1]  Quaternion=[1 0 0 0]  TranslationMethod=StandardAxis  TranslationCartesianOffset=[0 20 50]  TranslationCartesianOffsetUnits=mm  TranslationStandardAxis=-Y  TranslationStandardOffset=10  TranslationStandardOffsetUnits=mm  TranslationROffset=0  TranslationROffsetUnits=m  TranslationThetaOffset=0  TranslationThetaOffsetUnits=deg  TranslationZOffset=0  TranslationZOffsetUnits=m
  Rigid Transform6 : sm_lib/Frames and Transforms/Rigid Transform  RotationMethod=None  FollAlignAxisA=+X  BaseAlignAxisA=+Y  FollAlignAxisB=+Y  BaseAlignAxisB=+Z  RotationStandardAxis=+Z  RotationAngle=0  RotationAngleUnits=deg  RotationArbitraryAxis=[0 0 1]  RotationSequenceAxes=FollowerAxes  RotationSequence=XYX  RotationSequenceAngles=[0 0 0]  RotationSequenceAnglesUnits=deg  RotationMatrix=[1 0 0;0 1 0;0 0 1]  Quaternion=[1 0 0 0]  TranslationMethod=StandardAxis  TranslationCartesianOffset=[0 0 0]  TranslationCartesianOffsetUnits=m  TranslationStandardAxis=+Y  TranslationStandardOffset=20  TranslationStandardOffsetUnits=mm  TranslationROffset=0  TranslationROffsetUnits=m  TranslationThetaOffset=0  TranslationThetaOffsetUnits=deg  TranslationZOffset=0  TranslationZOffsetUnits=m
  Rigid Transform8 : sm_lib/Frames and Transforms/Rigid Transform  RotationMethod=None  FollAlignAxisA=+X  BaseAlignAxisA=+Y  FollAlignAxisB=+Y  BaseAlignAxisB=+Z  RotationStandardAxis=+Z  RotationAngle=0  RotationAngleUnits=deg  RotationArbitraryAxis=[0 0 1]  RotationSequenceAxes=FollowerAxes  RotationSequence=XYX  RotationSequenceAngles=[0 0 0]  RotationSequenceAnglesUnits=deg  RotationMatrix=[1 0 0;0 1 0;0 0 1]  Quaternion=[1 0 0 0]  TranslationMethod=StandardAxis  TranslationCartesianOffset=[0 0 0]  TranslationCartesianOffsetUnits=m  TranslationStandardAxis=-X  TranslationStandardOffset=225  TranslationStandardOffsetUnits=mm  TranslationROffset=0  TranslationROffsetUnits=m  TranslationThetaOffset=0  TranslationThetaOffsetUnits=deg  TranslationZOffset=0  TranslationZOffsetUnits=m
  Rigid Transform9 : sm_lib/Frames and Transforms/Rigid Transform  RotationMethod=None  FollAlignAxisA=+X  BaseAlignAxisA=+Y  FollAlignAxisB=+Y  BaseAlignAxisB=+Z  RotationStandardAxis=+Z  RotationAngle=0  RotationAngleUnits=deg  RotationArbitraryAxis=[0 0 1]  RotationSequenceAxes=FollowerAxes  RotationSequence=XYX  RotationSequenceAngles=[0 0 0]  RotationSequenceAnglesUnits=deg  RotationMatrix=[1 0 0;0 1 0;0 0 1]  Quaternion=[1 0 0 0]  TranslationMethod=StandardAxis  TranslationCartesianOffset=[0 0 0]  TranslationCartesianOffsetUnits=m  TranslationStandardAxis=+Z  TranslationStandardOffset=120  TranslationStandardOffsetUnits=mm  TranslationROffset=0  TranslationROffsetUnits=m  TranslationThetaOffset=0  TranslationThetaOffsetUnits=deg  TranslationZOffset=0  TranslationZOffsetUnits=m
  SixDOF1 : sm_lib/Joints/6-DOF Joint  JointMode=Normal  CompositeWrenchDir=FollowerOnBase  CompositeWrenchFrame=BaseFrame  SenseConstraintForce=off  SenseConstraintTorque=off  SenseTotalForce=off  SenseTotalTorque=off  PxPositionTargetSpecify=off  PxPositionTargetPriority=High  PxPositionTargetValue=0  PxPositionTargetValueUnits=m  PxVelocityTargetSpecify=off  PxVelocityTargetPriority=High  PxVelocityTargetValue=0  PxVelocityTargetValueUnits=m/s  PxEquilibriumPosition=0  PxEquilibriumPositionUnits=m  PxSpringStiffness=0  PxSpringStiffnessUnits=N/m  PxDampingCoefficient=0  PxDampingCoefficientUnits=N/(m/s)  PxLowerLimitSpecify=off  PxLowerLimitBound=-1  PxLowerLimitBoundUnits=m  PxLowerLimitStiffness=1e6  PxLowerLimitStiffnessUnits=N/m  PxLowerLimitDamping=1e3  PxLowerLimitDampingUnits=N/(m/s)  PxLowerLimitTransitionRegionWidth=1e-4  PxLowerLimitTransitionRegionWidthUnits=m  PxUpperLimitSpecify=off  PxUpperLimitBound=1  PxUpperLimitBoundUnits=m  PxUpperLimitStiffness=1e6  PxUpperLimitStiffnessUnits=N/m  PxUpperLimitDamping=1e3  PxUpperLimitDampingUnits=N/(m/s)  PxUpperLimitTransitionRegionWidth=1e-4  PxUpperLimitTransitionRegionWidthUnits=m  PxTorqueActuationMode=NoTorque  PxMotionActuationMode=ComputedMotion  PxSensePosition=off  PxSenseVelocity=off  PxSenseAcceleration=off  PxSenseTorqueForce=off  PxSenseLowerLimitTorqueForce=off  PxSenseUpperLimitTorqueForce=off  PyPositionTargetSpecify=on  PyPositionTargetPriority=High  PyPositionTargetValue=30  PyPositionTargetValueUnits=mm  PyVelocityTargetSpecify=off  PyVelocityTargetPriority=High  PyVelocityTargetValue=0  PyVelocityTargetValueUnits=m/s  PyEquilibriumPosition=0  PyEquilibriumPositionUnits=m  PySpringStiffness=0  PySpringStiffnessUnits=N/m  PyDampingCoefficient=0  PyDampingCoefficientUnits=N/(m/s)  PyLowerLimitSpecify=off  PyLowerLimitBound=-1  PyLowerLimitBoundUnits=m  PyLowerLimitStiffness=1e6  PyLowerLimitStiffnessUnits=N/m  PyLowerLimitDamping=1e3  PyLowerLimitDampingUnits=N/(m/s)  PyLowerLimitTransitionRegionWidth=1e-4  PyLowerLimitTransitionRegionWidthUnits=m  PyUpperLimitSpecify=off  PyUpperLimitBound=1  PyUpperLimitBoundUnits=m  PyUpperLimitStiffness=1e6  PyUpperLimitStiffnessUnits=N/m  PyUpperLimitDamping=1e3  PyUpperLimitDampingUnits=N/(m/s)  PyUpperLimitTransitionRegionWidth=1e-4  PyUpperLimitTransitionRegionWidthUnits=m  PyTorqueActuationMode=NoTorque  PyMotionActuationMode=ComputedMotion  PySensePosition=off  PySenseVelocity=off  PySenseAcceleration=off  PySenseTorqueForce=off  PySenseLowerLimitTorqueForce=off  PySenseUpperLimitTorqueForce=off  PzPositionTargetSpecify=off  PzPositionTargetPriority=High  PzPositionTargetValue=0  PzPositionTargetValueUnits=m  PzVelocityTargetSpecify=off  PzVelocityTargetPriority=High  PzVelocityTargetValue=0  PzVelocityTargetValueUnits=m/s  PzEquilibriumPosition=0  PzEquilibriumPositionUnits=m  PzSpringStiffness=0  PzSpringStiffnessUnits=N/m  PzDampingCoefficient=0  PzDampingCoefficientUnits=N/(m/s)  PzLowerLimitSpecify=off  PzLowerLimitBound=-1  PzLowerLimitBoundUnits=m  PzLowerLimitStiffness=1e6  PzLowerLimitStiffnessUnits=N/m  PzLowerLimitDamping=1e3  PzLowerLimitDampingUnits=N/(m/s)  PzLowerLimitTransitionRegionWidth=1e-4  PzLowerLimitTransitionRegionWidthUnits=m  PzUpperLimitSpecify=off  PzUpperLimitBound=1  PzUpperLimitBoundUnits=m  PzUpperLimitStiffness=1e6  PzUpperLimitStiffnessUnits=N/m  PzUpperLimitDamping=1e3  PzUpperLimitDampingUnits=N/(m/s)  PzUpperLimitTransitionRegionWidth=1e-4  PzUpperLimitTransitionRegionWidthUnits=m  PzTorqueActuationMode=NoTorque  PzMotionActuationMode=ComputedMotion  PzSensePosition=off  PzSenseVelocity=off  PzSenseAcceleration=off  PzSenseTorqueForce=off  PzSenseLowerLimitTorqueForce=off  PzSenseUpperLimitTorqueForce=off  SphPositionTargetSpecify=off  SphPositionTargetPriority=High  SphPositionTargetRotationMethod=None  SphPositionTargetFollAlignAxisA=+X  SphPositionTargetBaseAlignAxisA=+Y  SphPositionTargetFollAlignAxisB=+Y  SphPositionTargetBaseAlignAxisB=+Z  SphPositionTargetRotationStandardAxis=+Z  SphPositionTargetRotationAngle=0  SphPositionTargetRotationAngleUnits=deg  SphPositionTargetRotationArbitraryAxis=[0 0 1]  SphPositionTargetRotationSequenceAxes=FollowerAxes  SphPositionTargetRotationSequence=XYX  SphPositionTargetRotationSequenceAngles=[0 0 0]  SphPositionTargetRotationSequenceAnglesUnits=deg  SphPositionTargetRotationMatrix=[1 0 0;0 1 0;0 0 1]  SphPositionTargetQuaternion=[1 0 0 0]  SphVelocityTargetSpecify=off  SphVelocityTargetPriority=High  SphVelocityTargetValue=[0 0 0]  SphVelocityTargetValueUnits=deg/s  SphVelocityTargetInFollowerFrame=on  SphEqPosRotationMethod=None  SphEqPosFollAlignAxisA=+X  SphEqPosBaseAlignAxisA=+Y  SphEqPosFollAlignAxisB=+Y  SphEqPosBaseAlignAxisB=+Z  SphEqPosRotationStandardAxis=+Z  SphEqPosRotationAngle=0  SphEqPosRotationAngleUnits=deg  SphEqPosRotationArbitraryAxis=[0 0 1]  SphEqPosRotationSequenceAxes=FollowerAxes  SphEqPosRotationSequence=XYX  SphEqPosRotationSequenceAngles=[0 0 0]  SphEqPosRotationSequenceAnglesUnits=deg  SphEqPosRotationMatrix=[1 0 0;0 1 0;0 0 1]  SphEqPosQuaternion=[1 0 0 0]  SphSpringStiffness=0  SphSpringStiffnessUnits=N*m/deg  SphDampingCoefficient=0  SphDampingCoefficientUnits=N*m/(deg/s)  SphLowerLimitSpecify=off  SphLowerLimitBound=15  SphLowerLimitBoundUnits=deg  SphLowerLimitStiffness=1e4  SphLowerLimitStiffnessUnits=N*m/deg  SphLowerLimitDamping=10  SphLowerLimitDampingUnits=N*m/(deg/s)  SphLowerLimitTransitionRegionWidth=0.1  SphLowerLimitTransitionRegionWidthUnits=deg  SphUpperLimitSpecify=off  SphUpperLimitBound=45  SphUpperLimitBoundUnits=deg  SphUpperLimitStiffness=1e4  SphUpperLimitStiffnessUnits=N*m/deg  SphUpperLimitDamping=10  SphUpperLimitDampingUnits=N*m/(deg/s)  SphUpperLimitTransitionRegionWidth=0.1  SphUpperLimitTransitionRegionWidthUnits=deg  SphTorqueActuationMode=NoTorque  SphActuateTorqueX=off  SphActuateTorqueY=off  SphActuateTorqueZ=off  SphActuateTorque=off  SphActuationFrame=BaseFrame  SphSensePosition=off  SphSenseVelocityX=off  SphSenseVelocityY=off  SphSenseVelocityZ=off  SphSenseVelocity=off  SphSenseAccelerationX=off  SphSenseAccelerationY=off  SphSenseAccelerationZ=off  SphSenseAcceleration=off  SphSenseLowerLimitTorqueMag=off  SphSenseUpperLimitTorqueMag=off  SphSensingFrame=FollowerFrame
  Transform3 : sm_lib/Frames and Transforms/Rigid Transform  RotationMethod=ArbitraryAxis  FollAlignAxisA=+X  BaseAlignAxisA=+Y  FollAlignAxisB=+Y  BaseAlignAxisB=+Z  RotationStandardAxis=+Z  RotationAngle=smiData.RigidTransform(33).angle  RotationAngleUnits=rad  RotationArbitraryAxis=smiData.RigidTransform(33).axis  RotationSequenceAxes=FollowerAxes  RotationSequence=XYX  RotationSequenceAngles=[0 0 0]  RotationSequenceAnglesUnits=deg  RotationMatrix=[1 0 0;0 1 0;0 0 1]  Quaternion=[1 0 0 0]  TranslationMethod=Cartesian  TranslationCartesianOffset=smiData.RigidTransform(33).translation  TranslationCartesianOffsetUnits=mm  TranslationStandardAxis=+Z  TranslationStandardOffset=0  TranslationStandardOffsetUnits=m  TranslationROffset=0  TranslationROffsetUnits=m  TranslationThetaOffset=0  TranslationThetaOffsetUnits=deg  TranslationZOffset=0  TranslationZOffsetUnits=m
  StationaryPartsFrame : PMIOPort  Side=Left
  RotatingDisc : PMIOPort  Port=2  Side=Left
  Slot2Frame : PMIOPort  Port=3  Side=Left
  SortingAreaFrame : PMIOPort  Port=4  Side=Left
  PistonFrame : PMIOPort  Port=5  Side=Left
  PickupAreaFrame : PMIOPort  Port=6  Side=Left
  SuctionFrame : PMIOPort  Port=7  Side=Left
  " SuctionForce" : PMIOPort  Port=8  Side=Left
  Lid 1 : PMIOPort  Port=9  Side=Left
  Out1 : Outport
  Out2 : Outport  Port=2
  wires:
  Lid 1 with Pickup Area/1 -> Bus Selector1/1
  Lid 1 with Sorting Area/1 -> Bus Selector2/1
  Bus Selector2/1 -> Abs1/1  "<Normal Force>"
  Abs1/1 -> Data Type Conversion/1
  Relay/1 -> Out1/1
  Data Type Conversion/1 -> Relay/1
  Bus Selector1/1 -> Abs2/1  "<Normal Force>"
  Abs2/1 -> Data Type Conversion1/1
  Data Type Conversion1/1 -> Relay1/1
  Relay1/1 -> Out2/1
  connections:
  Lid 1 with Magazine Slot/RConn1 -- Slot2Frame/RConn1
  Transform3/LConn1 -- StationaryPartsFrame/RConn1
  Rigid Transform8/LConn1 -- RotatingDisc/RConn1 -- Rigid Transform9/LConn1
  Lid 1 with Sorting Area/RConn1 -- Rigid Transform9/RConn1 -- Lid 1 with Assembly Area/RConn1
  Lid 1 with Magazine Slot/LConn1 -- Rigid Transform6/RConn1 -- Lid 1 with Sorting Slot/LConn1
  Lid 1 with Magazine Surface/RConn1 -- Rigid Transform8/RConn1
  Rigid Transform11/LConn1 -- Rigid Transform4/LConn1 -- Rigid Transform3/LConn1 -- Rigid Transform2/LConn1 -- Rigid Transform6/LConn1 -- Rigid Transform1/LConn1 -- Product_Lid_stp_1_RIGID1/LConn1 -- SixDOF1/RConn1
  Rigid Transform/RConn1 -- Lid 1 with Sorting Slot/RConn1
  Transform3/RConn1 -- SixDOF1/LConn1
  " Lid 1 with Piston"/RConn1 -- PistonFrame/RConn1
  Rigid Transform3/RConn1 -- Lid 1 with Pickup Area/LConn1
  PickupAreaFrame/RConn1 -- Lid 1 with Pickup Area/RConn1
  Rigid Transform2/RConn1 -- " Lid 1 with Piston"/LConn1
  Rigid Transform4/RConn1 -- Lid 1 with Suction/LConn1 -- Internal Force/RConn1
  Lid 1 with Suction/RConn1 -- SuctionFrame/RConn1 -- Internal Force/LConn1
  Lid 1/RConn1 -- Rigid Transform11/RConn1
  " SuctionForce"/RConn1 -- Internal Force/LConn2
  Lid 1 with Magazine Surface/LConn1 -- Rigid Transform1/RConn1 -- Lid 1 with Sorting Area/LConn1 -- Lid 1 with Assembly Area/LConn1
  SortingAreaFrame/RConn1 -- Rigid Transform/LConn1
